simulink model "cp6_ej2_comp"  (R2026a)
settings: Solver=VariableStepAuto  StopTime=60  MaxStep=0.005
libraries: slpidlib x1
settings Model: Creator=benja  LastModifiedBy=benja

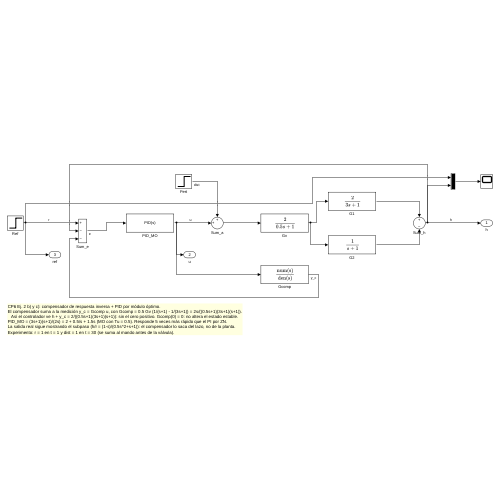
[thumbnail: Simulink's stored preview of the top-level diagram]
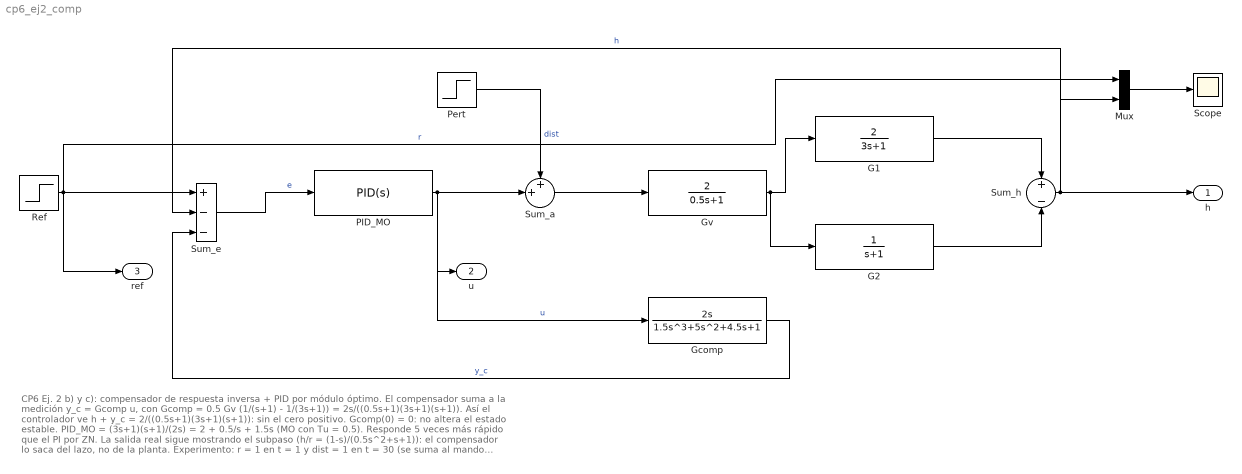
== system cp6_ej2_comp ==
  note: CP6 Ej. 2 b) y c): compensador de respuesta inversa + PID por módulo óptimo.
      | El compensador suma a la medición y_c = Gcomp u, con Gcomp = 0.5 Gv (1/(s+1) - 1/(3s+1)) = 2s/((0.5s+1)(3s+1)(s+1)).
      |    Así el controlador ve h + y_c = 2/((0.5s+1)(3s+1)(s+1)): sin el cero positivo. Gcomp(0) = 0: no altera el estado estable.
      | PID_MO = (3s+1)(s+1)/(2s) = 2 + 0.5/s + 1.5s (MO con Tu = 0.5). Responde 5 veces más rápido que el PI por ZN.
      | La salida real sigue mostrando el subpaso (h/r = (1-s)/(0.5s^2+s+1)): el compensador lo saca del lazo, no de la planta.
      | Experimento: r = 1 en t = 1 y dist = 1 en t = 30 (se suma al mando antes de la válvula).
  G1 : TransferFcn  Numerator=2  Denominator=[3 1]
  G2 : TransferFcn  Numerator=1  Denominator=[1 1]
  Gcomp : TransferFcn  Numerator=[2 0]  Denominator=[1.5 5 4.5 1]
  Gv : TransferFcn  Numerator=2  Denominator=[0.5 1]
  Mux : Mux  Inputs=2
  PID_MO : slpidlib/PID Controller  Controller=PID  Form=Parallel  TimeDomain=Continuous-time  UseExternalTs=off  SampleTime=-1  IntegratorMethod=Forward Euler  FilterMethod=Forward Euler  ControllerParametersSource=internal  P=2  I=0.5  UseKiTs=off  D=1.5  UseExternalDerivativeSource=off  N=20  UseFilter=on  TunerSelectOption=Transfer Function Based (PID Tuner App)  InitialConditionSource=internal  InitialConditionForIntegrator=0  InitialConditionForFilter=0  DifferentiatorICPrevScaledInput=0  ExternalReset=none  TrackingMode=off  Kt=1  LimitOutput=off  SatLimitsSource=internal  UpperSaturationLimit=inf  LowerSaturationLimit=-inf  LinearizeAsGain=on  AntiWindupMode=none  Kb=1  LimitIntegrator=off  UpperIntegratorSaturationLimit=inf  LowerIntegratorSaturationLimit=-inf  POutMin=[]  POutMax=[]  IOutMin=[]  IOutMax=[]  DOutMin=[]  DOutMax=[]  NOutMin=[]  NOutMax=[]  SumOutMin=[]  SumOutMax=[]  SaturationOutMin=[]  SaturationOutMax=[]  PParamMin=[]  PParamMax=[]  IParamMin=[]  IParamMax=[]  DParamMin=[]  DParamMax=[]  NParamMin=[]  NParamMax=[]  KbParamMin=[]  KbParamMax=[]  KtParamMin=[]  KtParamMax=[]  KbOutMin=[]  KbOutMax=[]  KtOutMin=[]  KtOutMax=[]  IntegratorOutMin=[]  IntegratorOutMax=[]  FilterOutMin=[]  FilterOutMax=[]  SumI1OutMin=[]  SumI1OutMax=[]  SumI2OutMin=[]  SumI2OutMax=[]  SumI3OutMin=[]  SumI3OutMax=[]  SumI4OutMin=[]  SumI4OutMax=[]  SumDOutMin=[]  SumDOutMax=[]  DifferentiatorOutMin=[]  DifferentiatorOutMax=[]  FilterDiffOutCoefMin=[]  FilterDiffOutCoefMax=[]  ReciprocalOutMin=[]  ReciprocalOutMax=[]  SumDenOutMin=[]  SumDenOutMax=[]  SumNumOutMin=[]  SumNumOutMax=[]  DivideOutMin=[]  DivideOutMax=[]  UdiffTsProdOutMin=[]  UdiffTsProdOutMax=[]  NTsProdOutMin=[]  NTsProdOutMax=[]  UintegralTsProdOutMin=[]  UintegralTsProdOutMax=[]  UngainTsProdOutMin=[]  UngainTsProdOutMax=[]  ClampingZeroOutDataTypeStr=Inherit: Inherit via back propagation  ClampingZeroOutMin=[]  ClampingZeroOutMax=[]  FilterDenConstantOutDataTypeStr=Inherit: Inherit via back propagation  FilterDenConstantOutMin=[]  FilterDenConstantOutMax=[]  PCopyOutDataTypeStr=Inherit: Inherit via back propagation  PCopyOutMin=[]  PCopyOutMax=[]  NCopyOutDataTypeStr=Inherit: Inherit via back propagation  NCopyOutMin=[]  NCopyOutMax=[]  IntegratorContinuousStateAttributes=''  IntegratorStateMustResolveToSignalObject=off  IntegratorRTWStateStorageClass=Auto  FilterContinuousStateAttributes=''  FilterStateMustResolveToSignalObject=off  FilterRTWStateStorageClass=Auto  ParallelPVariant=InternalParameters  IdealPVariant=Disabled  IVariant=InternalParameters  DVariant=InternalParameters  IntegratorVariant=Continuous  SatVariant=Disabled  AWVariant=Passthrough  PCopyVariant=Disabled  TRVariant=Disabled  FdbkBlocksVariant=Forward  IdealPFdbkVariant=Disabled  SatFdbkVariant=Disabled  DerivativeFilterVariant=ContFilter  NVariant=InternalParameters  NCopyVariant=Disabled  FilterICVariant=InternalICsFilter  IntegratorICVariant=InternalICs  ExternalResetVariant=Disabled  TRSumVariant=Passthrough  SumFdbkVariant=Disabled  SumVariant=Sum_PID  TsampFilterVariant=InternalTs  TsampNgainVariant=Passthrough  TsampIntegralVariant=Disabled_SignalSpec  ExternalSaturationOutDataTypeStr=Inherit: Same as second input  DerivativeSourceVariant=ErrorSignal  PreIntVariant=InternalPreInt
  Pert : Step  Time=30  SampleTime=0
  Ref : Step  SampleTime=0
  Scope : Scope
  Sum_a : Sum  Inputs=++|
  Sum_e : Sum  Inputs=+--
  Sum_h : Sum  Inputs=+|-
  h : Outport
  u : Outport  Port=2
  ref : Outport  Port=3
  wires:
  Ref/1 -> Sum_e/1, ref/1, Mux/1  "r"
  Sum_e/1 -> PID_MO/1  "e"
  PID_MO/1 -> Sum_a/2, u/1, Gcomp/1  "u"
  Pert/1 -> Sum_a/1  "dist"
  Sum_a/1 -> Gv/1
  Gv/1 -> G1/1, G2/1
  G1/1 -> Sum_h/1
  G2/1 -> Sum_h/2
  Sum_h/1 -> h/1, Sum_e/2, Mux/2  "h"
  Gcomp/1 -> Sum_e/3  "y_c"
  Mux/1 -> Scope/1
